simulink model "PC_model"  (R2026a)
settings: Solver=ode23  StopTime=10  MaxStep=1e-3
undefined symbols (not defined in the file): alpha1, alpha2, alpha3, alpha4, alpha5, c1, c2, c3, Fa, Fd, k0, k1, k2, k3, L, L1, m1, m2, m3, magnitude, v
libraries: simulink x1
settings Model: Creator=16915  LastModifiedBy=16915

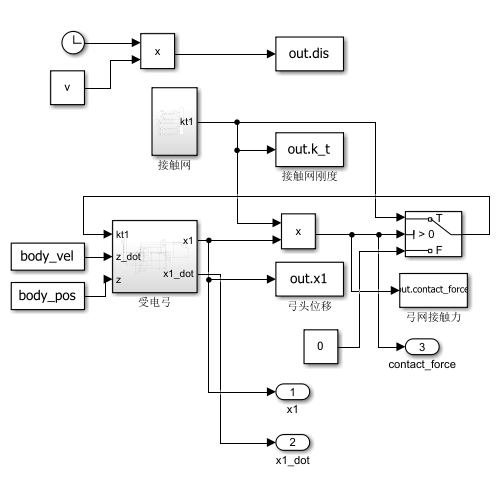
[thumbnail: Simulink's stored preview of the top-level diagram]
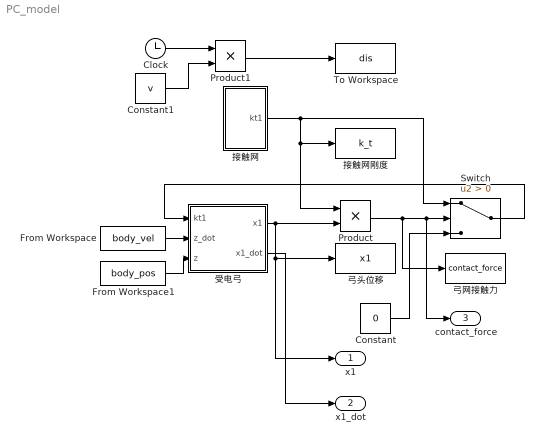
== system PC_model ==
  Clock : Clock
  Constant : Constant  Value=0
  Constant1 : Constant  Value=v
  From Workspace : FromWorkspace  VariableName=body_vel
  From Workspace1 : FromWorkspace  VariableName=body_pos
  Product : Product
  Product1 : Product
  Switch : Switch  Criteria=u2 > Threshold  SaturateOnIntegerOverflow=off  InputSameDT=off
  To Workspace : ToWorkspace  VariableName=dis  SaveFormat=Timeseries  SampleTime=-1
  受电弓 : Subsystem
  弓头位移 : ToWorkspace  VariableName=x1  SampleTime=1e-3
  弓网接触力 : ToWorkspace  VariableName=contact_force  SampleTime=1e-3
  接触网 : Subsystem
  接触网刚度 : ToWorkspace  VariableName=k_t  SampleTime=1e-3
  x1 : Outport
  x1_dot : Outport  Port=2
  contact_force : Outport  Port=3
  wires:
  Product/1 -> contact_force/1, Switch/2, 弓网接触力/1
  From Workspace1/1 -> 受电弓/3(z)
  Product1/1 -> To Workspace/1
  接触网/1(kt1) -> 接触网刚度/1, Product/1, Switch/1
  From Workspace/1 -> 受电弓/2(z_dot)
  Clock/1 -> Product1/1
  Constant1/1 -> Product1/2
  Switch/1 -> 受电弓/1(kt1)
  受电弓/2(x1_dot) -> x1_dot/1
  受电弓/1(x1) -> x1/1, 弓头位移/1, Product/2
  Constant/1 -> Switch/3

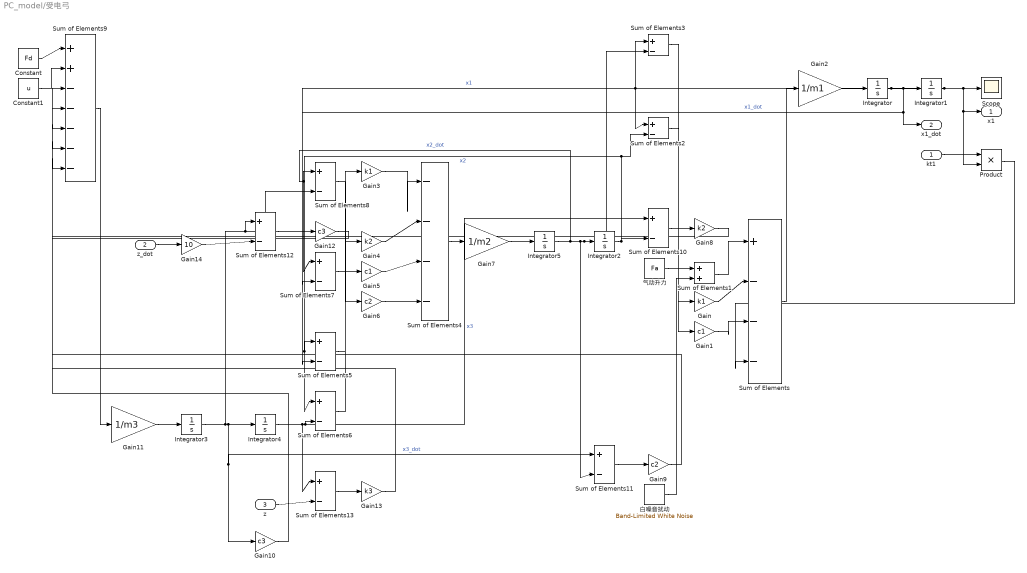
== system PC_model/受电弓 ==
  kt1 : Inport
  z_dot : Inport  Port=2
  z : Inport  Port=3
  Constant : Constant  Value=Fd
  Constant1 : Constant  Value=u
  Gain : Gain  Gain=k1
  Gain1 : Gain  Gain=c1
  Gain10 : Gain  Gain=c3
  Gain11 : Gain  Gain=1/m3
  Gain12 : Gain  Gain=c3
  Gain13 : Gain  Gain=k3
  Gain14 : Gain  Gain=10
  Gain2 : Gain  Gain=1/m1
  Gain3 : Gain  Gain=k1
  Gain4 : Gain  Gain=k2
  Gain5 : Gain  Gain=c1
  Gain6 : Gain  Gain=c2
  Gain7 : Gain  Gain=1/m2
  Gain8 : Gain  Gain=k2
  Gain9 : Gain  Gain=c2
  Integrator{,1..5} (6 alike) : Integrator
  Product : Product
  Scope : Scope
  Sum of Elements : Sum  Inputs=|+---
  Sum of Elements1 : Sum
  Sum of Elements{2..3,5..8,10..13} (10 alike) : Sum  Inputs=|+-
  Sum of Elements4 : Sum  Inputs=|----
  Sum of Elements9 : Sum  Inputs=|++-----|
  气动升力 : Constant  Value=Fa
  白噪音扰动 : simulink/Sources/Band-Limited White Noise  Cov=noise_coef  Ts=1e-3  seed=[23341]
  x1 : Outport
  x1_dot : Outport  Port=2
  wires:
  Gain1/1 -> Sum of Elements/3
  Constant/1 -> Sum of Elements9/1
  z_dot/1 -> Gain14/1
  z/1 -> Sum of Elements13/2
  Constant1/1 -> Sum of Elements9/2
  Sum of Elements9/1 -> Gain11/1
  Gain14/1 -> Sum of Elements12/2
  Gain2/1 -> Integrator/1
  Gain11/1 -> Integrator3/1
  Integrator3/1 -> Gain10/1, Sum of Elements11/1, Integrator4/1, Sum of Elements8/2, Sum of Elements12/1  "x3_dot"
  Sum of Elements1/1 -> Sum of Elements/1
  Sum of Elements10/1 -> Gain8/1
  Sum of Elements11/1 -> Gain9/1
  Sum of Elements12/1 -> Gain12/1
  Integrator/1 -> x1_dot/1, Sum of Elements7/2, Integrator1/1, Sum of Elements3/1  "x1_dot"
  Integrator4/1 -> Sum of Elements10/1, Sum of Elements6/2, Sum of Elements13/1  "x3"
  Gain10/1 -> Sum of Elements9/5
  Sum of Elements6/1 -> Gain4/1
  Sum of Elements5/1 -> Gain3/1
  Sum of Elements7/1 -> Gain5/1
  Sum of Elements8/1 -> Gain6/1
  Gain12/1 -> Sum of Elements9/6
  Sum of Elements2/1 -> Gain/1
  Sum of Elements3/1 -> Gain1/1
  Sum of Elements4/1 -> Gain7/1
  Sum of Elements13/1 -> Gain13/1
  Gain7/1 -> Integrator5/1
  Gain3/1 -> Sum of Elements4/1
  Gain4/1 -> Sum of Elements4/2
  Gain5/1 -> Sum of Elements4/3
  Gain6/1 -> Sum of Elements4/4
  Gain13/1 -> Sum of Elements9/7
  Integrator1/1 -> Sum of Elements2/1, Sum of Elements5/2, x1/1, Product/2, Scope/1  "x1"
  Integrator5/1 -> Integrator2/1, Sum of Elements3/2, Sum of Elements11/2, Sum of Elements7/1, Sum of Elements8/1  "x2_dot"
  Integrator2/1 -> Sum of Elements6/1, Sum of Elements5/1, Sum of Elements2/2, Sum of Elements10/2  "x2"
  气动升力/1 -> Sum of Elements1/1
  Gain9/1 -> Sum of Elements9/4
  白噪音扰动/1 -> Sum of Elements1/2
  Gain8/1 -> Sum of Elements9/3
  Gain/1 -> Sum of Elements/2
  Sum of Elements/1 -> Gain2/1
  kt1/1 -> Product/1
  Product/1 -> Sum of Elements/4

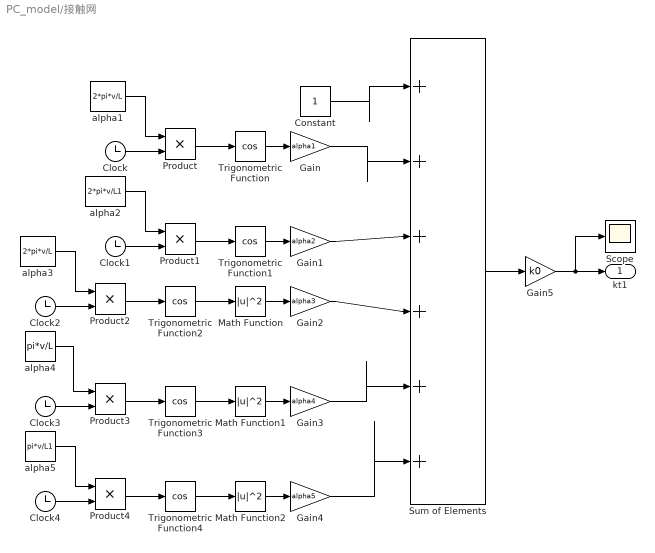
== system PC_model/接触网 ==
  Clock{,1..4} (5 alike) : Clock
  Constant : Constant
  Gain : Gain  Gain=alpha1
  Gain1 : Gain  Gain=alpha2
  Gain2 : Gain  Gain=alpha3
  Gain3 : Gain  Gain=alpha4
  Gain4 : Gain  Gain=alpha5
  Gain5 : Gain  Gain=k0
  Math Function : Math  Operator=magnitude^2
  Math Function1 : Math  Operator=magnitude^2
  Math Function2 : Math  Operator=magnitude^2
  Product{,1..4} (5 alike) : Product
  Scope : Scope
      settings: ActiveDisplayYMinimum=1462.8874669881548  ActiveDisplayYMaximum=5419.4744481124271
  Sum of Elements : Sum  Inputs=|++++++|
  Trigonometric Function{,1..4} (5 alike) : Trigonometry  Operator=cos
  alpha1 : Constant  Value=2*pi*v/L
  alpha2 : Constant  Value=2*pi*v/L1
  alpha3 : Constant  Value=2*pi*v/L
  alpha4 : Constant  Value=pi*v/L
  alpha5 : Constant  Value=pi*v/L1
  kt1 : Outport
  wires:
  alpha5/1 -> Product4/1
  alpha4/1 -> Product3/1
  alpha3/1 -> Product2/1
  Gain1/1 -> Sum of Elements/3
  Clock4/1 -> Product4/2
  Clock/1 -> Product/2
  Clock3/1 -> Product3/2
  Clock2/1 -> Product2/2
  Trigonometric Function2/1 -> Math Function/1
  alpha1/1 -> Product/1
  alpha2/1 -> Product1/1
  Constant/1 -> Sum of Elements/1
  Clock1/1 -> Product1/2
  Gain4/1 -> Sum of Elements/6
  Product/1 -> Trigonometric Function/1
  Product2/1 -> Trigonometric Function2/1
  Math Function2/1 -> Gain4/1
  Product1/1 -> Trigonometric Function1/1
  Product3/1 -> Trigonometric Function3/1
  Trigonometric Function1/1 -> Gain1/1
  Product4/1 -> Trigonometric Function4/1
  Sum of Elements/1 -> Gain5/1
  Trigonometric Function3/1 -> Math Function1/1
  Trigonometric Function4/1 -> Math Function2/1
  Trigonometric Function/1 -> Gain/1
  Math Function/1 -> Gain2/1
  Math Function1/1 -> Gain3/1
  Gain/1 -> Sum of Elements/2
  Gain2/1 -> Sum of Elements/4
  Gain3/1 -> Sum of Elements/5
  Gain5/1 -> kt1/1, Scope/1
